simulink library "Lib_Piccolo"  (R2018b)
settings: Solver=VariableStepAuto  StartTime=0.0  StopTime=10.0  RelTol=1e-3
values from neighbouring files (symbols this model uses):
  AccelErrInt2Brakes = 0.15    [SimulationControlConfig16P.m]    (also in SimulationControlConfig16P_LEGACY.m; SimulationControlConfigTAILLESS.m = 0.2; SimulationControlConfigUTAIL.m = 0.2)
  AileronMax = 25    [SimulationControlConfig16P.m]    (also in SimulationControlConfig16P_LEGACY.m; SimulationControlConfigTAILLESS.m; SimulationControlConfigUTAIL.m)
  AileronPower = 0.00268    [SimulationControlConfig16P.m]    (also in SimulationControlConfig16P_LEGACY.m; SimulationControlConfigTAILLESS.m; SimulationControlConfigUTAIL.m)
  AileronSurfaceMax = 45    [SimulationControlConfig16P.m]    (also in SimulationControlConfig16P_LEGACY.m)
  AileronTrim = 0    [SimulationControlConfig16P.m]    (also in SimulationControlConfig16P_LEGACY.m; SimulationControlConfigTAILLESS.m; SimulationControlConfigUTAIL.m)
  Alt = 1000 + TerrainHeight    [SimulationStateConfig.m]
  AltCruise_m = testPlans(testIndx).terrainElevation * 0.3048 + 200    [SimulationControlConfig16P.m]    (also in SimulationControlConfigTAILLESS.m = 1083; SimulationControlConfigUTAIL.m = testPlans(testIndx).terrainElevation * 0.3048 + 152)
  AltitudeRate2PitchCmdIntegratorInit = 0.1    [SimulationControlPre.m]
  AltMax = 10000    [SimulationControlConfig16P.m]    (also in SimulationControlConfig16P_LEGACY.m; SimulationControlConfigTAILLESS.m; SimulationControlConfigUTAIL.m)
  AltMaxAccel = 1.25    [SimulationControlConfig16P.m]    (also in SimulationControlConfig16P_LEGACY.m = 0.9; SimulationControlConfigTAILLESS.m = 1.7; SimulationControlConfigUTAIL.m = 2)
  AltMin = 0    [SimulationControlConfig16P.m]    (also in SimulationControlConfig16P_LEGACY.m; SimulationControlConfigTAILLESS.m; SimulationControlConfigUTAIL.m)
  AltRateCmd2Pitch = 0.50    (= 0.5)    [SimulationControlConfig16P.m]    (also in SimulationControlConfig16P_LEGACY.m = 0.6; SimulationControlConfigTAILLESS.m = 0.2; SimulationControlConfigUTAIL.m = 0.3)
  AltRateError2Pitch = 0.40    (= 0.4)    [SimulationControlConfig16P.m]    (also in SimulationControlConfig16P_LEGACY.m; SimulationControlConfigTAILLESS.m = 0.55; SimulationControlConfigUTAIL.m = 0.55)
  AltRateErrorInt2Pitch = 0.50    (= 0.5)    [SimulationControlConfig16P.m]    (also in SimulationControlConfig16P_LEGACY.m = 0.45; SimulationControlConfigTAILLESS.m; SimulationControlConfigUTAIL.m = 0.75)
  AltRateLpfCutOff = 3    [SimulationControlConfig16P.m]    (also in SimulationControlConfig16P_LEGACY.m; SimulationControlConfigTAILLESS.m = 2; SimulationControlConfigUTAIL.m = 2)
  AutoNosegear2Rudder = 26    [SimulationControlConfig16P.m]    (also in SimulationControlConfig16P_LEGACY.m; SimulationControlConfigTAILLESS.m = 25.2; SimulationControlConfigUTAIL.m = 14)
  b = 5.54    [SimulationControlConfig16P.m]    (also in SimulationControlConfig16P_LEGACY.m; SimulationControlConfigTAILLESS.m = 2.37; SimulationControlConfigUTAIL.m = 2.37)
  Bank2AileronIntegratorInit = 0    [SimulationControlPre.m]
  BankMax_User = BankMax_User/180*pi    (= 0.523598775598)    [SimulationControlConfig16P.m]    (also in SimulationControlConfig16P_LEGACY.m; SimulationControlConfigTAILLESS.m = 0.610865238198; SimulationControlConfigUTAIL.m = 0.628318530718)
  baseLegFlaps = 20    [SimulationControlConfig16P.m]    (also in SimulationControlConfig16P_LEGACY.m = 0; SimulationControlConfigTAILLESS.m = 15; SimulationControlConfigUTAIL.m = 10)
  C = GeneticOpt.C    [SimulationCostFunction.m]
  c = Sw/b    (= 0.841696750903)    [SimulationControlConfig16P.m]    (also in SimulationControlConfig16P_LEGACY.m; SimulationControlConfigTAILLESS.m = 0.354008438819; SimulationControlConfigUTAIL.m = 0.354008438819)
  cell2WheelFactorMG = 5.98    [SimulationSensorConfig16P_LEGACY.m]
  cell2WheelFactorNG = 1    [SimulationSensorConfig16P_LEGACY.m]
  cellSatMaxMG = 15000    [SimulationSensorConfig16P.m]    (also in SimulationSensorConfig16P_LEGACY.m; SimulationSensorConfigTAILLESS7P.m; SimulationSensorConfigUTAIL7P.m)
  cellSatMaxNG = 1000    [SimulationSensorConfig16P.m]    (also in SimulationSensorConfig16P_LEGACY.m; SimulationSensorConfigTAILLESS7P.m; SimulationSensorConfigUTAIL7P.m)
  cellSatMinMG = -15000    [SimulationSensorConfig16P.m]    (also in SimulationSensorConfig16P_LEGACY.m; SimulationSensorConfigTAILLESS7P.m; SimulationSensorConfigUTAIL7P.m)
  cellSatMinNG = -1000    [SimulationSensorConfig16P.m]    (also in SimulationSensorConfig16P_LEGACY.m; SimulationSensorConfigTAILLESS7P.m; SimulationSensorConfigUTAIL7P.m)
  CL_Limit = CL_Max    (= 0.54)    [SimulationControlConfig16P.m]    (also in SimulationControlConfig16P_LEGACY.m; SimulationControlConfigTAILLESS.m; SimulationControlConfigUTAIL.m = 0.53)
  CL_Max = 0.54    [SimulationControlConfig16P.m]    (also in SimulationControlConfig16P_LEGACY.m; SimulationControlConfigTAILLESS.m; SimulationControlConfigUTAIL.m = 0.53)
  CL_Max_Nom = 0.465    [SimulationControlConfig16P.m]    (also in SimulationControlConfig16P_LEGACY.m; SimulationControlConfigTAILLESS.m = 0.39; SimulationControlConfigUTAIL.m)
  CL_Min = 0    [SimulationControlConfig16P.m]    (also in SimulationControlConfig16P_LEGACY.m; SimulationControlConfigTAILLESS.m; SimulationControlConfigUTAIL.m)
  ClimbMaxFraction = 0.35    [SimulationControlConfig16P.m]    (also in SimulationControlConfig16P_LEGACY.m = 0.24; SimulationControlConfigTAILLESS.m = 0.19; SimulationControlConfigUTAIL.m = 0.21)
  ClimboutMaxBank = 7.0    (= 7)    [SimulationControlConfig16P.m]    (also in SimulationControlConfig16P_LEGACY.m; SimulationControlConfigTAILLESS.m = 5; SimulationControlConfigUTAIL.m)
  ClimboutTimer = 7.0    (= 7)    [SimulationControlConfig16P.m]    (also in SimulationControlConfig16P_LEGACY.m; SimulationControlConfigTAILLESS.m; SimulationControlConfigUTAIL.m)
  dCl_per_dFlap = 0.005581818    [SimulationControlConfig16P.m]    (also in SimulationControlConfig16P_LEGACY.m = 0; SimulationControlConfigTAILLESS.m = 0; SimulationControlConfigUTAIL.m = 0)
  DecelerationCmd = 3.1    [SimulationControlConfig16P.m]    (also in SimulationControlConfig16P_LEGACY.m; SimulationControlConfigTAILLESS.m = 0.1; SimulationControlConfigUTAIL.m = 0.1)
  DeRotateLogicEndTimer = abs((NoseDownLimit_Deg-1)/DeRotateRamp_Dps)    [SimulationControlConfig16P.m]    (also in SimulationControlConfig16P_LEGACY.m; SimulationControlConfigTAILLESS.m; SimulationControlConfigUTAIL.m)
  DeRotateLogicHoldNoseUpTimer = 0.1    [SimulationControlConfig16P.m]    (also in SimulationControlConfig16P_LEGACY.m; SimulationControlConfigTAILLESS.m; SimulationControlConfigUTAIL.m)
  DeRotateLogicTimerTimeout = 2    [SimulationControlConfig16P.m]    (also in SimulationControlConfig16P_LEGACY.m; SimulationControlConfigTAILLESS.m; SimulationControlConfigUTAIL.m)
  DeRotateLowerCmdSaturation = 0    [SimulationControlConfig16P.m]    (also in SimulationControlConfig16P_LEGACY.m; SimulationControlConfigTAILLESS.m; SimulationControlConfigUTAIL.m)
  DeRotateRamp_Dps = 3    [SimulationControlConfig16P.m]    (also in SimulationControlConfig16P_LEGACY.m; SimulationControlConfigTAILLESS.m = 8; SimulationControlConfigUTAIL.m = 8)
  DeRotateUpperCmdSaturation = 7    [SimulationControlConfig16P.m]    (also in SimulationControlConfig16P_LEGACY.m; SimulationControlConfigTAILLESS.m; SimulationControlConfigUTAIL.m)
  DescentMaxFraction = 0.22    [SimulationControlConfig16P.m]    (also in SimulationControlConfig16P_LEGACY.m = 0.2; SimulationControlConfigTAILLESS.m = 0.17; SimulationControlConfigUTAIL.m = 0.17)
  DesktopSimTerrainOffset_m = 0.406    [SimulationAircraftConfig.m]
  downwindFlaps = 0    [SimulationControlConfig16P.m]    (also in SimulationControlConfig16P_LEGACY.m; SimulationControlConfigTAILLESS.m; SimulationControlConfigUTAIL.m)
  DP_init = 0.5*1.225*V_init^2    [SimulationControlConfig16P.m]    (also in SimulationControlConfig16P_LEGACY.m; SimulationControlConfigTAILLESS.m; SimulationControlConfigUTAIL.m)
  dscNoiseMG = 1    [SimulationSensorConfig16P_LEGACY.m]
  dscNoiseNG = 0.25    [SimulationSensorConfig16P_LEGACY.m]
  DSCnumBits = 24    [SimulationSensorConfig16P.m]    (also in SimulationSensorConfig16P_LEGACY.m; SimulationSensorConfigTAILLESS7P.m; SimulationSensorConfigUTAIL7P.m)
  DSCRangeMaxMG = 15000    [SimulationSensorConfig16P.m]    (also in SimulationSensorConfig16P_LEGACY.m; SimulationSensorConfigTAILLESS7P.m; SimulationSensorConfigUTAIL7P.m)
  DSCRangeMaxNG = 1000    [SimulationSensorConfig16P.m]    (also in SimulationSensorConfig16P_LEGACY.m; SimulationSensorConfigTAILLESS7P.m; SimulationSensorConfigUTAIL7P.m)
  DSCRangeMinMG = -15000    [SimulationSensorConfig16P.m]    (also in SimulationSensorConfig16P_LEGACY.m; SimulationSensorConfigTAILLESS7P.m; SimulationSensorConfigUTAIL7P.m)
  DSCRangeMinNG = -1000    [SimulationSensorConfig16P.m]    (also in SimulationSensorConfig16P_LEGACY.m; SimulationSensorConfigTAILLESS7P.m; SimulationSensorConfigUTAIL7P.m)
  dt = DLLSim.dt    [SimulationTimeStep.m]    (also in SimulationTrim.m = 0.02)
  EarlyTouchdownThreshold = 3.0    (= 3)    [SimulationControlConfig16P.m]    (also in SimulationControlConfig16P_LEGACY.m; SimulationControlConfigTAILLESS.m = 2.2; SimulationControlConfigUTAIL.m = 2.5)
  ElevatorDeflectionRate = 15    [SimulationControlConfig16P.m]    (also in SimulationControlConfig16P_LEGACY.m = 12; SimulationControlConfigTAILLESS.m = 10; SimulationControlConfigUTAIL.m = 12)
  ElevatorMax = 25    [SimulationControlConfig16P.m]    (also in SimulationControlConfig16P_LEGACY.m; SimulationControlConfigTAILLESS.m; SimulationControlConfigUTAIL.m)
  ElevatorPower = -0.002209    [SimulationControlConfig16P.m]    (also in SimulationControlConfig16P_LEGACY.m; SimulationControlConfigTAILLESS.m = -0.002956; SimulationControlConfigUTAIL.m = -0.00205983)
  ElevatorTrim = -3.5    [SimulationControlConfig16P.m]    (also in SimulationControlConfig16P_LEGACY.m; SimulationControlConfigTAILLESS.m = -6; SimulationControlConfigUTAIL.m = -8)
  elevonBias = 0    [SimulationControlConfig16P.m]    (also in SimulationControlConfig16P_LEGACY.m; SimulationControlConfigTAILLESS.m; SimulationControlConfigUTAIL.m)
  Enable_TAS_Protection = 0    [SimulationControlConfig16P.m]    (also in SimulationControlConfig16P_LEGACY.m; SimulationControlConfigTAILLESS.m; SimulationControlConfigUTAIL.m)
  EnableCrossTrackAbort = 1    [SimulationControlConfig16P.m]    (also in SimulationControlConfigTAILLESS.m; SimulationControlConfigUTAIL.m)
  EnergyBandwidth = 0.02    [SimulationControlConfig16P.m]    (also in SimulationControlConfig16P_LEGACY.m; SimulationControlConfigTAILLESS.m = 0.06; SimulationControlConfigUTAIL.m = 0.06)
  EngineLhFuelCut = 0    [SimulationAircraftConfig.m]
  EngineRhFuelCut = 0    [SimulationAircraftConfig.m]
  FastThrottleRate = 0.075    [SimulationControlConfig16P.m]    (also in SimulationControlConfig16P_LEGACY.m = 0.05; SimulationControlConfigTAILLESS.m = 0.1; SimulationControlConfigUTAIL.m = 0.1)
  FilterWarmUpTime = 2    [SimulationSensorConfig16P.m]    (also in SimulationSensorConfig16P_LEGACY.m; SimulationSensorConfigTAILLESS7P.m; SimulationSensorConfigUTAIL7P.m)
  finalApproachFlaps = 20    [SimulationControlConfig16P.m]    (also in SimulationControlConfig16P_LEGACY.m = 0; SimulationControlConfigTAILLESS.m = 22; SimulationControlConfigUTAIL.m = 10)
  FinalDescentSlope_Deg = testPlans(testIndx).descentSlope    [SimulationControlConfig16P.m]    (also in SimulationControlConfig16P_LEGACY.m; SimulationControlConfigTAILLESS.m; SimulationControlConfigUTAIL.m)
  flapMax = 0    [SimulationControlConfig16P.m]    (also in SimulationControlConfig16P_LEGACY.m; SimulationControlConfigTAILLESS.m; SimulationControlConfigUTAIL.m)
  flapRate = 7.5    [SimulationControlConfig16P.m]    (also in SimulationControlConfig16P_LEGACY.m; SimulationControlConfigTAILLESS.m = 6.6; SimulationControlConfigUTAIL.m)
  FlareHeight = 5    [SimulationControlConfig16P.m]    (also in SimulationControlConfig16P_LEGACY.m = 4.8; SimulationControlConfigTAILLESS.m = 2.5; SimulationControlConfigUTAIL.m = 2)
  FlareVerticalRate_mps = -0.4    [SimulationControlConfig16P.m]    (also in SimulationControlConfig16P_LEGACY.m = -0.5; SimulationControlConfigTAILLESS.m = -0.15; SimulationControlConfigUTAIL.m = -0.15)
  Fp_Aileron = 0.55*2*pi*RollRateLpfCutoff*dt    [SimulationControlConfig16P.m]    (also in SimulationControlConfig16P_LEGACY.m; SimulationControlConfigTAILLESS.m; SimulationControlConfigUTAIL.m)
  Fp_Alt = 0.55*AltBandwidth    (= 0.099)    [SimulationControlConfig16P.m]    (also in SimulationControlConfig16P_LEGACY.m; SimulationControlConfigTAILLESS.m = 0.587477826221; SimulationControlConfigUTAIL.m = 0.69115038379)
  Fp_AltRate = 0.55*2*pi*AltRateLpfCutOff*dt    [SimulationControlConfig16P.m]    (also in SimulationControlConfig16P_LEGACY.m; SimulationControlConfigTAILLESS.m; SimulationControlConfigUTAIL.m)
  Fp_Elevator = 0.55*2*pi*PitchRateLpfCutoff*dt    [SimulationControlConfig16P.m]    (also in SimulationControlConfig16P_LEGACY.m; SimulationControlConfigTAILLESS.m; SimulationControlConfigUTAIL.m)
  Fp_Energy = 0.55*2*pi*EnergyBandwidth    (= 0.069115038379)    [SimulationControlConfig16P.m]    (also in SimulationControlConfig16P_LEGACY.m; SimulationControlConfigTAILLESS.m = 0.207345115137; SimulationControlConfigUTAIL.m = 0.207345115137)
  Fp_Energy2 = 0.55*2*pi*EnergyBandwidth*dt    [SimulationControlConfig16P.m]    (also in SimulationControlConfig16P_LEGACY.m; SimulationControlConfigTAILLESS.m; SimulationControlConfigUTAIL.m)
  Fp_Pitch = 0.55*2*pi*PitchBandwidth    (= 2.76460153516)    [SimulationControlConfig16P.m]    (also in SimulationControlConfig16P_LEGACY.m = 3.11017672705; SimulationControlConfigTAILLESS.m = 3.80132711084; SimulationControlConfigUTAIL.m = 2.41902634326)
  Fp_Pitch_2 = 0.55*2*pi*PitchBandwidth*dt    [SimulationControlConfig16P.m]    (also in SimulationControlConfig16P_LEGACY.m; SimulationControlConfigTAILLESS.m; SimulationControlConfigUTAIL.m)
  Fp_Roll = RollBandwidth^2    (= 1)    [SimulationControlConfig16P.m]    (also in SimulationControlConfig16P_LEGACY.m = 1.44; SimulationControlConfigTAILLESS.m; SimulationControlConfigUTAIL.m)
  Fp_Rudder = 0.55*2*pi*YawRateLpfCutoff*dt    [SimulationControlConfig16P.m]    (also in SimulationControlConfig16P_LEGACY.m; SimulationControlConfigTAILLESS.m; SimulationControlConfigUTAIL.m)
  Fp_TAS = 0.55*2*pi*TASBandwidth    (= 0.103672557568)    [SimulationControlConfig16P.m]    (also in SimulationControlConfig16P_LEGACY.m; SimulationControlConfigTAILLESS.m = 0.172787595947; SimulationControlConfigUTAIL.m = 0.172787595947)
  Fp_TAS_Filter = 2*pi*TasLpfCutoff*dt    [SimulationControlConfig16P.m]    (also in SimulationControlConfig16P_LEGACY.m; SimulationControlConfigTAILLESS.m; SimulationControlConfigUTAIL.m)
  Fp_Turn = 0.55*2*pi*TurnErrLPFcutoff    (= 0.0345575191895)    [SimulationControlConfig16P.m]    (also in SimulationControlConfig16P_LEGACY.m; SimulationControlConfigTAILLESS.m = 0.172787595947; SimulationControlConfigUTAIL.m = 0.172787595947)
  Fp_TurnDerr = 0.55*2*pi*TurnDerivativeLPFcutoff    (= 0.0345575191895)    [SimulationControlConfig16P.m]    (also in SimulationControlConfig16P_LEGACY.m; SimulationControlConfigTAILLESS.m = 0.172787595947; SimulationControlConfigUTAIL.m = 0.172787595947)
  FTV = 3    [SimulationAircraftConfig.m]
  ftvStaticPositionError = 1/1.18    (= 0.847457627119)    [SimulationSensorConfig16P.m]    (also in SimulationSensorConfig16P_LEGACY.m; SimulationSensorConfigTAILLESS7P.m = 1; SimulationSensorConfigUTAIL7P.m = 1)
  g = 9.81    [SimulationStateConfig.m]
  GustSpd_Kts = testPlans(testIndx).gustSpd    [SimulationStateConfig.m]
  GustTriggerVal = testPlans(testIndx).gustTriggerVal    [SimulationStateConfig.m]
  HeadingErr2TurnRate = 0.5    [SimulationControlConfig16P.m]    (also in SimulationControlConfig16P_LEGACY.m; SimulationControlConfigTAILLESS.m; SimulationControlConfigUTAIL.m)
  HeadingErrDer2TurnRate = 0.3    [SimulationControlConfig16P.m]    (also in SimulationControlConfig16P_LEGACY.m; SimulationControlConfigTAILLESS.m; SimulationControlConfigUTAIL.m)
  IASbounce = IASstall*0.8    [SimulationControlPre.m]
  IAScruiseCMD = sqrt(2*m*9.81/(1.225*Sw*CL_cruise))    [SimulationControlConfig16P.m]    (also in SimulationControlConfig16P_LEGACY.m; SimulationControlConfigTAILLESS.m; SimulationControlConfigUTAIL.m)
  IASfinalCMD = 1.12 * IASmin    [SimulationControlConfig16P.m]    (also in SimulationControlConfig16P_LEGACY.m = 1.10 * IASmin; SimulationControlConfigTAILLESS.m = 1.10 * IASmin; SimulationControlConfigUTAIL.m = 1.15 * IASmin)
  IASflareCMD = IASstall    [SimulationControlConfig16P.m]    (also in SimulationControlConfig16P_LEGACY.m; SimulationControlConfigTAILLESS.m; SimulationControlConfigUTAIL.m)
  IASmax = 64    [SimulationControlConfig16P.m]    (also in SimulationControlConfig16P_LEGACY.m = 46; SimulationControlConfigTAILLESS.m = 38.58; SimulationControlConfigUTAIL.m = 35)
  IASmin = sqrt(2*m*9.81/(1.225*Sw*0.9*CL_Max_Nom))    [SimulationControlConfig16P.m]    (also in SimulationControlConfig16P_LEGACY.m; SimulationControlConfigTAILLESS.m; SimulationControlConfigUTAIL.m)
  IASshortCMD = IASstall    [SimulationControlConfig16P.m]    (also in SimulationControlConfig16P_LEGACY.m; SimulationControlConfigTAILLESS.m; SimulationControlConfigUTAIL.m)
  IASstall = sqrt(2*m*9.81/(1.225*Sw*CL_Max))    [SimulationControlConfig16P.m]    (also in SimulationControlConfig16P_LEGACY.m; SimulationControlConfigTAILLESS.m; SimulationControlConfigUTAIL.m)
  inFlight = 1    [SimulationControlConfig16P.m]    (also in SimulationControlConfigTAILLESS.m; SimulationControlConfigUTAIL.m)
  JetCatOffset = 5    [SimulationControlConfig16P.m]    (also in SimulationControlConfig16P_LEGACY.m)
  LaunchRollingElevator = -1.5    [SimulationControlConfig16P.m]    (also in SimulationControlConfig16P_LEGACY.m; SimulationControlConfigTAILLESS.m = 1; SimulationControlConfigUTAIL.m = 1)
  ldg_NosegearMax = 10    [SimulationControlConfig16P.m]    (also in SimulationControlConfig16P_LEGACY.m; SimulationControlConfigTAILLESS.m; SimulationControlConfigUTAIL.m)
  ldg_TrackVyErrInt2Nosegear = 0.1250    (= 0.125)    [SimulationControlConfig16P.m]    (also in SimulationControlConfig16P_LEGACY.m; SimulationControlConfigTAILLESS.m = 0.00714285714286; SimulationControlConfigUTAIL.m = 0.00714285714286)
  ldg_TrackVyErrPro2Nosegear = 0.35    [SimulationControlConfig16P.m]    (also in SimulationControlConfig16P_LEGACY.m; SimulationControlConfigTAILLESS.m = 0.0546666666667; SimulationControlConfigUTAIL.m = 0.0546666666667)
  ldg_TrackY2Vy = 0.07    [SimulationControlConfig16P.m]    (also in SimulationControlConfig16P_LEGACY.m; SimulationControlConfigTAILLESS.m = 0.17; SimulationControlConfigUTAIL.m = 0.17)
  ldg_Vy2NosegearScalingPower = 1.075    [SimulationControlConfig16P.m]    (also in SimulationControlConfig16P_LEGACY.m; SimulationControlConfigTAILLESS.m = 0.6; SimulationControlConfigUTAIL.m = 0.5)
  ldg_Y2VyScalingPower = 0.175    [SimulationControlConfig16P.m]    (also in SimulationControlConfig16P_LEGACY.m; SimulationControlConfigTAILLESS.m = 0; SimulationControlConfigUTAIL.m = 0)
  ldg_YawRate2Nosegear = 0.175    [SimulationControlConfig16P.m]    (also in SimulationControlConfig16P_LEGACY.m; SimulationControlConfigTAILLESS.m = 0.065; SimulationControlConfigUTAIL.m = 0.065)
  LiftSlope = 0.064285    [SimulationControlConfig16P.m]    (also in SimulationControlConfig16P_LEGACY.m; SimulationControlConfigTAILLESS.m = 0.058631; SimulationControlConfigUTAIL.m)
  LPFaileronInit = 0    [SimulationControlPre.m]
  LPFclestInit = 0    [SimulationControlPre.m]
  LPFenergyFFInit = 0    [SimulationControlPre.m]
  LPFtasInit = V_init + 2    [SimulationControlPre.m]
  LPFthrottleInit = ThrottleTrim    [SimulationControlPre.m]
  LPFturnErrInit = 0    [SimulationControlPre.m]
  ... (+115 more)
undefined symbols (not defined in the file or in its folder): abortFlag, alphaHPF, apmDelay, BRWNOUT, CRAWOR, CRAWUR, DiscIntNeverNeededParam, DLLSim, DLLSimStep, ECOMOR, ECOMUR, Fp_Tas, GustTrigger_HeightAgl_m, IPSTAT, LCINTEG, Ldg_Persist_Time, LOWER_FLAGS, MSG_ENABLE, NoiseStd, OLDVAL, OVERRIDE_ENABLE, OVERRIDE_VALUE, REBOOT, reversionEnable, revIASMax, revIASMin, revPitchMax, revPitchMin, revPitchRateMax, revRollMax, revRollRateMax, SAMPLE, SCALON, SensorModel, sigbuilder_block, Sim_Vx, Sim_Vy, Sim_Vz, Sim_Xpos, Sim_Ypos, Sim_Zpos, SYSOR, SYSUR, TARE, TEMPOR, TEMPUR, testIndx, testPlan, testPlans, Trim_piccoloInCmd, Trim_REFSI_FD_IN_nmodeCgShifterCmd_Ft, Trim_REFSI_FD_IN_nmodeFlapLhIBCmd_Deg, Trim_REFSI_FD_IN_nmodeFlapLhOBCmd_Deg, Trim_REFSI_FD_IN_nmodeFlapRhIBCmd_Deg, Trim_REFSI_FD_IN_nmodeFlapRhOBCmd_Deg, Trim_REFSI_FD_IN_nmodeSlatLhCmd_Deg, Trim_REFSI_FD_IN_nmodeSlatRhCmd_Deg, Trim_REFSI_FD_IN_nmodeSplrLhInbdCmd_Deg, Trim_REFSI_FD_IN_nmodeSplrLhOutbdCmd_Deg ... (+5)
libraries: simulink x866, aerolibconvert2 x60, $bdroot x52, aerolibatmos2 x5, dspswit3 x5, simulink_extras x4, dsparch4 x2, Lib_Piccolo_Alt x2, eeGeneralControl x1, dspindex x1
(part 13 of 44)

== system Lib_Piccolo/Pitch to Elevator/LPF Elevator ==
  Input : Inport
  Reset : Inport  Port=2
  ResetValue : Inport  Port=3
  Add1 : Sum  Inputs=++|
  Compare To Constant2 : simulink/Logic and Bit Operations/Compare To Constant  relop=>  const=0  OutDataTypeStr=uint8
  Constant11 : Constant  Value=PitchRateLpfCutoff
  Switch : Switch  Criteria=u2 > Threshold
  Switch1 : Switch  Criteria=u2 > Threshold
  Unit Delay1 : UnitDelay  InitialCondition=LPFvRate2PitchInit*pi/180  SampleTime=-1
  a1 : Gain  Gain=1-Fp_Elevator
  b0 : Gain  Gain=Fp_Elevator
  Output : Outport
  wires:
  ResetValue/1 -> Switch/1
  Reset/1 -> Switch/2
  Switch/1 -> Unit Delay1/1
  Input/1 -> b0/1, Switch1/3
  Add1/1 -> Switch1/1, Switch/3
  b0/1 -> Add1/2
  Unit Delay1/1 -> a1/1
  a1/1 -> Add1/1
  Switch1/1 -> Output/1
  Compare To Constant2/1 -> Switch1/2
  Constant11/1 -> Compare To Constant2/1

== system Lib_Piccolo/Pitch to Elevator/Pitch Moment Caused By Damping ==
  note: An estimation of damping moment produced proportionally to body pitch rate.
  PitchRate_Body : Inport
  TAS : Inport  Port=2
  AverageWingChord : Constant  Value=c
  Constant : Constant  Value=PitchDamping
  Gain : Gain  Gain=2
  Multiply : Product  Inputs=***/
  DAMP : Outport
  wires:
  PitchRate_Body/1 -> Multiply/2
  TAS/1 -> Gain/1
  Constant/1 -> Multiply/1
  Multiply/1 -> DAMP/1
  Gain/1 -> Multiply/4
  AverageWingChord/1 -> Multiply/3

== system Lib_Piccolo/Pitch to Elevator/Reference Frame Conversion and Pitch Rate Limit Determination ==
  PitchCmd_Euler : Inport
  Pitch_Euler : Inport  Port=2
  Roll_Euler : Inport  Port=3
  V : Inport  Port=4
  Q : Inport  Port=5
  AeroVsStruct_Limit : Subsystem
  Constant : Constant  Value=PitchRateMax_User
  MATLAB Function : MATLAB Function  TreatAsAtomicUnit=on
  Saturation : Saturate  UpperLimit=100  LowerLimit=5
  Terminator : Terminator
  Terminator1 : Terminator
  PitchCmd_Body : Outport
  "Pitch_Body " : Outport  Port=2
  "Scalar " : Outport  Port=3
  PitchRateCmd_Body : Outport  Port=4
  "PitchRateLimit_Max " : Outport  Port=5
  "PitchRateLimit_Min " : Outport  Port=6
  wires:
  MATLAB Function/8(nPrime_Min) -> Terminator1/1
  MATLAB Function/7(nPrime_Max) -> Terminator/1
  Q/1 -> AeroVsStruct_Limit/1(Q)
  AeroVsStruct_Limit/2("nMin ") -> MATLAB Function/6(nMin)
  AeroVsStruct_Limit/1(nMax) -> MATLAB Function/5(nMax)
  MATLAB Function/4(PitchRateCmd_Body) -> PitchRateCmd_Body/1
  Constant/1 -> MATLAB Function/7(PitchRateMax_User)
  MATLAB Function/6(PitchRateLimit_Min) -> "PitchRateLimit_Min "/1
  MATLAB Function/5(PitchRateLimit_Max) -> "PitchRateLimit_Max "/1
  MATLAB Function/3(Scalar) -> "Scalar "/1
  MATLAB Function/2(Pitch_Body) -> "Pitch_Body "/1
  MATLAB Function/1(PitchCmd_Body) -> PitchCmd_Body/1
  Roll_Euler/1 -> MATLAB Function/3(Roll_Euler)
  Pitch_Euler/1 -> MATLAB Function/2(Pitch_Euler)
  PitchCmd_Euler/1 -> MATLAB Function/1(PitchCmd_Euler)
  V/1 -> Saturation/1
  Saturation/1 -> MATLAB Function/4(V)

== system Lib_Piccolo/Pitch to Elevator/TASLimit ==
  note: TAS saturates at ~ 100mps which in IAS is 6125Pa
  apMode : Inport
  <V_mps> : Inport  Port=2
  Compare To Constant1 : simulink/Logic and Bit Operations/Compare To Constant  relop=>=  const=5  OutDataTypeStr=uint8
  Compare To Constant2 : simulink/Logic and Bit Operations/Compare To Constant  relop=>=  const=11  OutDataTypeStr=uint8
  Compare To Constant4 : simulink/Logic and Bit Operations/Compare To Constant  relop=>=  const=10  OutDataTypeStr=uint8
  Gain : Gain  Gain=0.8
  Latch : Subsystem
  Saturation Dynamic1 : simulink/Discontinuities/Saturation Dynamic  OutMin=[]  OutMax=[]  OutDataTypeStr=Inherit: Same as second input  OutDataType=fixdt(1, 16)  OutScaling=2^-10  DoSatur=off
  Switch1 : Switch  Criteria=u2 > Threshold
  Switch2 : Switch  Criteria=u2 > Threshold
  TASmax : Constant  Value=100
  Out1 : Outport
  wires:
  TASmax/1 -> Saturation Dynamic1/1
  Gain/1 -> Switch2/1  "IASbounce"
  Compare To Constant1/1 -> Latch/2(Enable/!Rst)
  Switch1/1 -> Switch2/3
  apMode/1 -> Compare To Constant4/1, Compare To Constant2/1, Compare To Constant1/1
  Compare To Constant2/1 -> Latch/1(D)
  Latch/1(Q_Latched) -> Switch2/2
  <V_mps>/1 -> Saturation Dynamic1/2
  [IASmin] -> Switch1/3
  Saturation Dynamic1/1 -> Out1/1
  [IASstall] -> Switch1/1, Gain/1
  Compare To Constant4/1 -> Switch1/2
  Switch2/1 -> Saturation Dynamic1/3

== system Lib_Piccolo/Pitch to Elevator/Triggered Subsystem ==
  In1 : Inport
  Trigger : TriggerPort  TriggerType=falling  VariantControl=Variant
  Out1 : Outport
  wires:
  In1/1 -> Out1/1

== system Lib_Piccolo/Pitch to Elevator/resetCondition ==
  Compare To Constant1 : simulink/Logic and Bit Operations/Compare To Constant  relop=<=  const=2  OutDataTypeStr=uint8
  Compare To Constant3 : simulink/Logic and Bit Operations/Compare To Constant  relop===  const=11  OutDataTypeStr=uint8
  NOT : Logic  Operator=NOT  IconShape=distinctive  AllPortsSameDT=off  OutDataTypeStr=boolean
  OR : Logic  Operator=OR  Inputs=3  IconShape=distinctive  AllPortsSameDT=off  OutDataTypeStr=boolean
  reset : Outport
  wires:
  NOT/1 -> OR/3
  [ApGlobal] -> NOT/1
  Compare To Constant1/1 -> OR/2
  OR/1 -> reset/1  "Sim.KI_Pitch_Reset"
  Compare To Constant3/1 -> OR/1
  [Pic_AP_Mode] -> Compare To Constant3/1, Compare To Constant1/1

== system Lib_Piccolo/Pitch to Elevator/resetVal ==
  note: This init value is intended to aid trimming at start of in-flight simulation and should not be used for reset during liftoffs/bouncing. Will use 0 as alternative reset value as was done previously
  Constant1 : Constant  Value=Pitch2ElevatorIntegratorInit
  Constant2 : Constant  Value=0
  Constant3 : Constant  Value=0
  Switch : Switch  Threshold=9
  Switch1 : Switch  Threshold=3
  resetVal : Outport
  wires:
  Constant3/1 -> Switch1/3
  Switch1/1 -> Switch/3
  Constant1/1 -> Switch1/1
  Switch/1 -> resetVal/1
  [Pic_AP_Mode] -> Switch/2, Switch1/2
  Constant2/1 -> Switch/1

== system Lib_Piccolo/REF INS Replay/Slope Vz Calculation ==
  VGround : Inport
  apMode : Inport  Port=2
  Compare To Constant : simulink/Logic and Bit Operations/Compare To Constant  relop=>=  const=5  OutDataTypeStr=boolean
  Compare To Constant1 : simulink/Logic and Bit Operations/Compare To Constant  relop=>=  const=9  OutDataTypeStr=boolean
  Constant13 : Constant  Value=FinalDescentSlope_Deg*pi/180
  Constant14 : Constant  Value=ShortDescentSlope_Deg*pi/180
  CruiseSlope_Deg : Constant  Value=0
  Gain : Gain  Gain=-1
  Multiply10 : Product
  Sin3 : Trigonometry
  Switch3 : Switch  Criteria=u2 > Threshold
  Switch4 : Switch  Criteria=u2 > Threshold
  Vz_Cmd : Outport
  wires:
  Compare To Constant/1 -> Switch4/2
  Compare To Constant1/1 -> Switch3/2
  Switch4/1 -> Sin3/1
  Gain/1 -> Multiply10/1
  Constant13/1 -> Switch3/3
  VGround/1 -> Gain/1
  CruiseSlope_Deg/1 -> Switch4/3
  Multiply10/1 -> Vz_Cmd/1
  Constant14/1 -> Switch3/1
  Sin3/1 -> Multiply10/2
  Switch3/1 -> Switch4/1
  apMode/1 -> Compare To Constant1/1, Compare To Constant/1

== system Lib_Piccolo/Steering Controller Landing/Nosegear rudder mixer  ==
  "Desired nosegear " : Inport
  NoseGear2Rudder : Gain  Gain=AutoNosegear2Rudder
  Saturation : Saturate  UpperLimit=ldg_NosegearMax  LowerLimit=-ldg_NosegearMax
  Saturation1 : Saturate  UpperLimit=RudderMax  LowerLimit=-RudderMax
  rad2deg : Gain  Gain=180/pi
  Nosegear command : Outport
  Rudder command : Outport  Port=2
  wires:
  rad2deg/1 -> Saturation/1, NoseGear2Rudder/1
  "Desired nosegear "/1 -> rad2deg/1
  NoseGear2Rudder/1 -> Saturation1/1
  Saturation/1 -> Nosegear command/1
  Saturation1/1 -> Rudder command/1

== system Lib_Piccolo/Steering Controller Landing/Nosegear scaling based on ground speed ==
  Ground Speed : Inport
  "Vy to nosegear scaling " : Inport  Port=2
  Divide : Product  Inputs=*/
  SteeringArm : Constant  Value=SteeringArm
  Vy Scalar1 : Math  Operator=pow  SaturateOnIntegerOverflow=on
  nosegear scalar : Outport
  wires:
  "Vy to nosegear scaling "/1 -> Vy Scalar1/2
  Divide/1 -> nosegear scalar/1
  SteeringArm/1 -> Divide/1
  Vy Scalar1/1 -> Divide/2
  Ground Speed/1 -> Vy Scalar1/1

== system Lib_Piccolo/Steering Controller Landing/Vy scaling based on ground speed ==
  Ground Speed : Inport
  Y to Vy scaling power : Inport  Port=2
  Power Function : Math  Operator=pow  SaturateOnIntegerOverflow=on
  Vy Scalar : Outport
  wires:
  Y to Vy scaling power/1 -> Power Function/2
  Ground Speed/1 -> Power Function/1
  Power Function/1 -> Vy Scalar/1

== system Lib_Piccolo/Steering Controller Transition/Nosegear rudder mixer  ==
  "Desired nosegear " : Inport
  NoseGear2Rudder : Gain  Gain=AutoNosegear2Rudder
  Saturation : Saturate  UpperLimit=NosegearMax  LowerLimit=-NosegearMax
  Saturation1 : Saturate  UpperLimit=RudderMax  LowerLimit=-RudderMax
  rad2deg : Gain  Gain=180/pi
  Nosegear command : Outport
  Rudder command : Outport  Port=2
  wires:
  rad2deg/1 -> Saturation/1, NoseGear2Rudder/1
  "Desired nosegear "/1 -> rad2deg/1
  NoseGear2Rudder/1 -> Saturation1/1
  Saturation/1 -> Nosegear command/1
  Saturation1/1 -> Rudder command/1

== system Lib_Piccolo/Steering Controller Transition/Nosegear scaling based on ground speed ==
  Ground Speed : Inport
  "Vy to nosegear scaling " : Inport  Port=2
  Divide : Product  Inputs=*/
  SteeringArm : Constant  Value=SteeringArm
  Vy Scalar1 : Math  Operator=pow  SaturateOnIntegerOverflow=on
  nosegear scalar : Outport
  wires:
  "Vy to nosegear scaling "/1 -> Vy Scalar1/2
  Divide/1 -> nosegear scalar/1
  SteeringArm/1 -> Divide/1
  Vy Scalar1/1 -> Divide/2
  Ground Speed/1 -> Vy Scalar1/1

== system Lib_Piccolo/Steering Controller Transition/Vy scaling based on ground speed ==
  Ground Speed : Inport
  Y to Vy scaling power : Inport  Port=2
  Power Function : Math  Operator=pow  SaturateOnIntegerOverflow=on
  Vy Scalar : Outport
  wires:
  Y to Vy scaling power/1 -> Power Function/2
  Ground Speed/1 -> Power Function/1
  Power Function/1 -> Vy Scalar/1

== system Lib_Piccolo/Throttle Control (Airspeed Mode)/1st Order Reference Model ==
  Pcmd : Inport
  Vcmd : Inport  Port=2
  Pact : Inport  Port=3
  "V " : Inport  Port=4
  Constant : Constant  Value=0
  Gain : Gain  Gain=Fp_Energy
  Gain3 : Gain  Gain=m*g
  Gain4 : Gain  Gain=m*g
  Saturation Dynamic : simulink/Discontinuities/Saturation Dynamic  OutMin=[]  OutMax=[]  OutDataTypeStr=Inherit: Same as second input  OutDataType=fixdt(1, 16)  OutScaling=2^-10  DoSatur=off
  Scope : Scope
  Subsystem : Subsystem
  Sum : Sum  Inputs=|+-
  Sum1 : Sum  Inputs=|++
  Rf : Outport
  wires:
  Saturation Dynamic/1 -> Rf/1  "Rf"
  Pcmd/1 -> Sum/1
  Pact/1 -> Sum/2
  Sum/1 -> Scope/1, Gain/1
  Gain/1 -> Sum1/2
  Sum1/1 -> Saturation Dynamic/2
  Constant/1 -> Sum1/1
  Vcmd/1 -> Subsystem/2(Vcmd)
  Subsystem/2("hdotMin ") -> Gain4/1
  Subsystem/1(hdotMax) -> Gain3/1
  "V "/1 -> Subsystem/1(V)
  Gain3/1 -> Saturation Dynamic/1
  Gain4/1 -> Saturation Dynamic/3

== system Lib_Piccolo/Throttle Control (Airspeed Mode)/Subsystem ==
  Throttle In : Inport
  Reset LPF : Inport  Port=2
  LPF Throttle Alpha : Subsystem
  Throttle Out : Outport
  wires:
  LPF Throttle Alpha/1(Output) -> Throttle Out/1  "TLA"
  Reset LPF/1 -> LPF Throttle Alpha/2(Reset)
  Throttle In/1 -> LPF Throttle Alpha/1(Input)  "TLA_Prefilter"

== system Lib_Piccolo/Throttle Control (Alt Mode)/1st Order Reference Model ==
  Pcmd : Inport
  Pact : Inport  Port=2
  "V " : Inport  Port=3
  Constant : Constant  Value=0
  Gain : Gain  Gain=Fp_Energy
  Gain1 : Gain  Gain=m*TASRateMax
  Gain2 : Gain  Gain=-1
  Saturation Dynamic : simulink/Discontinuities/Saturation Dynamic  OutMin=[]  OutMax=[]  OutDataTypeStr=Inherit: Same as second input  OutDataType=fixdt(1, 16)  OutScaling=2^-10  DoSatur=off
  Sum : Sum  Inputs=|+-
  Sum1 : Sum  Inputs=|++
  TEC Ref Max Rate Limit : Subsystem  Commented=on
  Rf : Outport
  wires:
  Saturation Dynamic/1 -> Rf/1  "Rf"
  Pcmd/1 -> Sum/1
  Pact/1 -> Sum/2
  Sum/1 -> Gain/1
  Gain/1 -> Sum1/2
  Sum1/1 -> Saturation Dynamic/2
  Gain1/1 -> Saturation Dynamic/1, Gain2/1
  Gain2/1 -> Saturation Dynamic/3
  Constant/1 -> Sum1/1
  "V "/1 -> Gain1/1

== system Lib_Piccolo/Throttle Control (Alt Mode)/Filter and Throttle Cut ==
  note: If IASFlareCMD equal 0 and Piccolo in Flare State Set Engine to Idle
  note: Set Engine To Idle After Touchdown
  Throttle In : Inport
  Reset LPF : Inport  Port=2
  apMode : Inport  Port=3
  Throttle Ramp In : Inport  Port=4
  AND : Logic  IconShape=distinctive  AllPortsSameDT=off  OutDataTypeStr=boolean
  Compare To Constant1 : simulink/Logic and Bit Operations/Compare To Constant  relop=>=  const=10  OutDataTypeStr=boolean
  Compare To Constant2 : simulink/Logic and Bit Operations/Compare To Constant  relop=>=  const=11  OutDataTypeStr=boolean
  Compare To Constant3 : simulink/Logic and Bit Operations/Compare To Constant  relop=<=  const=3  OutDataTypeStr=boolean
  Compare To Constant4 : simulink/Logic and Bit Operations/Compare To Constant  relop===  const=0  OutDataTypeStr=boolean
  Constant8 : Constant  Value=-ThrottleRateMax
  Constant9 : Constant  Value=IASflareCMD
  Discrete-Time Integrator1 : DiscreteIntegrator  ExternalReset=rising  InitialConditionSource=external  SampleTime=-1  LimitOutput=on  UpperSaturationLimit=ThrottleMax  LowerSaturationLimit=ThrottleMin  ICPrevOutput=DiscIntNeverNeededParam  ICPrevScaledInput=DiscIntNeverNeededParam
  LPF Throttle Alpha : Subsystem
  OR : Logic  Operator=OR  IconShape=distinctive  AllPortsSameDT=off  OutDataTypeStr=boolean
  OR1 : Logic  Operator=OR  IconShape=distinctive  AllPortsSameDT=off  OutDataTypeStr=boolean
  Switch : Switch  Criteria=u2 > Threshold
  Switch1 : Switch  Criteria=u2 > Threshold
  Switch8 : Switch  Criteria=u2 > Threshold
  Unit Delay : UnitDelay  SampleTime=-1
  Throttle Out : Outport
  wires:
  Compare To Constant4/1 -> AND/2
  Compare To Constant1/1 -> AND/1
  OR/1 -> Discrete-Time Integrator1/2, Switch8/2, Switch1/2, OR1/2
  AND/1 -> OR/1
  Constant9/1 -> Compare To Constant4/1
  Switch8/1 -> Throttle Out/1  "TLA"
  Throttle In/1 -> Switch1/3  "TLA_PreFilter"
  Compare To Constant2/1 -> OR/2
  Reset LPF/1 -> OR1/1
  apMode/1 -> Compare To Constant2/1, Compare To Constant3/1, Compare To Constant1/1
  LPF Throttle Alpha/1(Output) -> Switch/3, Switch8/3  "TLA_Postfilter"
  Constant8/1 -> Discrete-Time Integrator1/1
  Discrete-Time Integrator1/1 -> Switch8/1, Switch1/1  "Sim.TLA_Ramp"
  OR1/1 -> LPF Throttle Alpha/2(Reset)
  Switch1/1 -> LPF Throttle Alpha/1(Input)  "TLA"
  Throttle Ramp In/1 -> Switch/1
  Unit Delay/1 -> Discrete-Time Integrator1/3
  Compare To Constant3/1 -> Switch/2
  Switch/1 -> Unit Delay/1

== system Lib_Piccolo/Throttle Control (Alt Mode)/Flare Throttle Modifications 2 ==
  Throttle In (0 - 100%) : Inport
  Piccolo Elevator In (deg.) : Inport  Port=2
  AP Mode (0 - 12) : Inport  Port=3
  ApGlobal In : Inport  Port=4
  RTOActive In : Inport  Port=5
  EngineKill In : Inport  Port=6
  AND : Logic  Inputs=3  IconShape=distinctive  AllPortsSameDT=off  OutDataTypeStr=boolean
  AND1 : Logic  IconShape=distinctive  AllPortsSameDT=off  OutDataTypeStr=boolean
  Compare To Constant : simulink/Logic and Bit Operations/Compare To Constant  relop=>=  const=10  OutDataTypeStr=boolean
  Compare To Constant1 : simulink/Logic and Bit Operations/Compare To Constant  relop=>=  const=11  OutDataTypeStr=boolean
  Compare To Constant2 : simulink/Logic and Bit Operations/Compare To Constant  relop===  const=11  OutDataTypeStr=boolean
  Compare To Constant3 : simulink/Logic and Bit Operations/Compare To Constant  relop=>=  const=RolloutElevTrigger  OutDataTypeStr=boolean
  Compare To Constant4 : simulink/Logic and Bit Operations/Compare To Constant  relop=>=  const=9  OutDataTypeStr=boolean
  Constant : Constant  Value=useFlareSlew
  Constant1 : Constant  Value=ThrottleMaxFlare
  Constant2 : Constant  Value=ThrottleMinRollout
  Constant3 : Constant  Value=ThrottleMinFlare
  Constant4 : Constant  Value=useElevatorKill
  Constant5 : Constant  Value=ThrottleRateRever
  Constant6 : Constant  Value=ThrottleRateRollout
  Constant7 : Constant  Value=ThrottleRateFlare
  Gain5 : Gain  Gain=-1
  Latch : Subsystem
  NOT1 : Logic  Operator=NOT  IconShape=distinctive  AllPortsSameDT=off  OutDataTypeStr=boolean
  OR : Logic  Operator=NOR  Inputs=3  IconShape=distinctive  AllPortsSameDT=off  OutDataTypeStr=boolean
  Rate Limiter : Subsystem
  Saturation Dynamic : simulink/Discontinuities/Saturation Dynamic  OutMin=[]  OutMax=[]  OutDataTypeStr=Inherit: Same as second input  OutDataType=fixdt(1, 16)  OutScaling=2^-10  DoSatur=off
  Switch{,1..5} (6 alike) : Switch  Criteria=u2 > Threshold
  Throttle Out : Outport
  wires:
  Constant2/1 -> Switch5/1, Switch/1
  Throttle In (0 - 100%)/1 -> Switch5/3, Switch3/3
  Switch5/1 -> Saturation Dynamic/2
  RTOActive In/1 -> OR/2
  ApGlobal In/1 -> NOT1/1
  OR/1 -> AND/3
  NOT1/1 -> OR/1
  Switch1/1 -> AND1/2
  Compare To Constant2/1 -> Switch1/3, AND1/1
  Switch4/1 -> Rate Limiter/1(up), Gain5/1  "OverridenTECSlewRate"
  AND/1 -> Switch3/2, Rate Limiter/4(Enable)  "flareSlewActive"
  Saturation Dynamic/1 -> Rate Limiter/2(u)
  Constant/1 -> AND/1
  Gain5/1 -> Rate Limiter/3(lo)
  Compare To Constant/1 -> AND/2
  AP Mode (0 - 12)/1 -> Compare To Constant/1, Compare To Constant4/1, Compare To Constant1/1, Compare To Constant2/1
  Switch3/1 -> Throttle Out/1
  Constant1/1 -> Saturation Dynamic/1
  Constant3/1 -> Switch/3
  Switch/1 -> Saturation Dynamic/3
  Piccolo Elevator In (deg.)/1 -> Compare To Constant3/1
  AND1/1 -> Switch5/2, Switch/2
  Constant4/1 -> Switch1/2
  Compare To Constant3/1 -> Switch1/1
  Rate Limiter/1(Y) -> Switch3/1
  Compare To Constant1/1 -> Switch4/2, Latch/1(D)
  Constant7/1 -> Switch2/3
  Constant6/1 -> Switch4/1
  Compare To Constant4/1 -> Latch/2(Enable/!Rst)
  Latch/1(Q_Latched) -> Switch2/2
  Constant5/1 -> Switch2/1
  Switch2/1 -> Switch4/3
  EngineKill In/1 -> OR/3

== system Lib_Piccolo/Throttle Control (Alt Mode)/LPF Energy Alpha ==
  Input : Inport
  Reset : Inport  Port=2
  Add1 : Sum  Commented=on  Inputs=++|
  Compare To Constant1 : simulink/Logic and Bit Operations/Compare To Constant  relop=>  const=0  OutDataTypeStr=uint8
  Compare To Constant2 : simulink/Logic and Bit Operations/Compare To Constant  Commented=on  relop=>  const=0  OutDataTypeStr=uint8
  Constant : Constant  Value=dt
  Constant1 : Constant  Value=EnergyBandwidth
  Constant11 : Constant  Commented=on  Value=EnergyBandwidth
  LPF Alpha Energy : MATLAB Function  TreatAsAtomicUnit=on
  Memory1 : Memory  InitialCondition=LPFenergyFFInit  InheritSampleTime=on  LinearizeAsDelay=on
  Switch1 : Switch  Commented=on  Criteria=u2 > Threshold
  Switch2 : Switch  Criteria=u2 > Threshold
  Unit Delay1 : UnitDelay  Commented=on  InitialCondition=LPFenergyFFInit  SampleTime=-1
  a1 : Gain  Commented=on  Gain=1-Fp_Energy2
  b0 : Gain  Commented=on  Gain=Fp_Energy2
  Output : Outport
  wires:
  Constant1/1 -> LPF Alpha Energy/4(bandwidth), Compare To Constant1/1
  Memory1/1 -> LPF Alpha Energy/1(xFiltOld)
  LPF Alpha Energy/1(xFilt) -> Switch2/1, Memory1/1
  Compare To Constant1/1 -> Switch2/2
  Input/1 -> Switch2/3, LPF Alpha Energy/3(xNew)
  Switch2/1 -> Output/1
  Constant/1 -> LPF Alpha Energy/2(dt)
  Unit Delay1/1 -> a1/1
  b0/1 -> Add1/2
  Compare To Constant2/1 -> Switch1/2
  a1/1 -> Add1/1
  Constant11/1 -> Compare To Constant2/1
  Add1/1 -> Switch1/1, Unit Delay1/1

== system Lib_Piccolo/Throttle Control (Alt Mode)/O//L Throttle Ramp ==
  Feedback Bus : Inport
  startFlag : Inport  Port=2
  Bus Selector : BusSelector  OutputSignals=Sim_VGround
  Constant : Constant  Value=0
  Constant4 : Constant  Value=ThrottleMax
  Constant5 : Constant  Value=SlowThrottleRate
  Constant6 : Constant  Value=FastThrottleRate
  Integrator1 : Integrator  ExternalReset=rising  InitialCondition=PrelaunchThrottle
  Switch : Switch  Criteria=u2 > Threshold
  Switch2 : Switch  Criteria=u2 > Threshold  Threshold=ThrottleSwitchSpeed
  Switch3 : Switch  Threshold=ThrottleMax
  Sim.LaunchThrottleCmd : Outport
  wires:
  Integrator1/1 -> Switch3/3, Switch3/2  "throttleIntegrator"
  Constant6/1 -> Switch2/1
  Switch3/1 -> Switch/1  "throttleSat"
  Constant4/1 -> Switch3/1
  Switch2/1 -> Integrator1/1
  Constant5/1 -> Switch2/3
  Bus Selector/1 -> Switch2/2  "<Sim_VGround>"
  Feedback Bus/1 -> Bus Selector/1
  startFlag/1 -> Integrator1/2, Switch/2  "throttleflag"
  Switch/1 -> Sim.LaunchThrottleCmd/1
  Constant/1 -> Switch/3

== system Lib_Piccolo/Throttle Control (Alt Mode)/Reset Conditions ==
  AP Mode : Inport
  Compare To Constant1 : simulink/Logic and Bit Operations/Compare To Constant  relop=<=  const=3.0  OutDataTypeStr=boolean
  NOT : Logic  Operator=NOT  IconShape=distinctive  AllPortsSameDT=off  OutDataTypeStr=boolean
  OR : Logic  Operator=OR  Inputs=3  IconShape=distinctive  AllPortsSameDT=off  OutDataTypeStr=boolean
  Reset : Outport
  wires:
  NOT/1 -> OR/1
  [Flag_TAS_Priority] -> OR/2
  Compare To Constant1/1 -> OR/3
  [ApGlobal] -> NOT/1
  OR/1 -> Reset/1
  AP Mode/1 -> Compare To Constant1/1

== system Lib_Piccolo/Throttle Control (Alt Mode)/Speed Flags ==
  Feedback Bus : Inport
  AND : Logic  IconShape=distinctive  AllPortsSameDT=off  OutDataTypeStr=boolean
  AND1 : Logic  IconShape=distinctive  AllPortsSameDT=off  OutDataTypeStr=boolean
  Bus Selector : BusSelector  OutputSignals=V_mps,apMode
  CAS2TAS : Subsystem
  CAS2TAS1 : Subsystem
  Compare To Constant : simulink/Logic and Bit Operations/Compare To Constant  relop=>=  const=4  OutDataTypeStr=boolean
  Constant : Constant  Value=IASmin
  Constant6 : Constant  Value=IASmax
  Less Than : RelationalOperator  Operator=<  OutDataTypeStr=boolean  RndMeth=Simplest
  Less Than1 : RelationalOperator  Operator=>  OutDataTypeStr=boolean  RndMeth=Simplest
  Flag_Underspeed : Outport
  Flag_Overspeed : Outport  Port=2
  wires:
  Bus Selector/2 -> Compare To Constant/1  "<apMode>"
  Bus Selector/1 -> Less Than1/1, Less Than/1  "<V_mps>"
  Less Than/1 -> AND/1
  CAS2TAS/1(TAS) -> Less Than/2
  Constant/1 -> CAS2TAS/2(CAS)
  Constant6/1 -> CAS2TAS1/2(CAS)
  CAS2TAS1/1(TAS) -> Less Than1/2
  Less Than1/1 -> AND1/2
  Feedback Bus/1 -> Bus Selector/1, CAS2TAS1/1(Feedback Bus), CAS2TAS/1(Feedback Bus)
  AND/1 -> Flag_Underspeed/1  "Flag_Underspeed"
  AND1/1 -> Flag_Overspeed/1  "Flag_Overspeed"
  Compare To Constant/1 -> AND1/1, AND/2

== system Lib_Piccolo/VRate Reference Selection/Alt Max Accel Rate Limit ==
  note: Y(k)
  note: U(k)
  up : Inport
  u : Inport  Port=2
  lo : Inport  Port=3
  Delay Input2 : UnitDelay  Description=Store in Global RAM  DisableCoverage=on  InitialCondition=RateLimitAltAccelInit  SampleTime=-1
  Difference Inputs1 : Sum  Description=Add in CPU  DisableCoverage=on  Inputs=+-  OutDataTypeStr=Inherit: Inherit via back propagation
  Difference Inputs2 : Sum  Description=Add in CPU  OutDataTypeStr=Inherit: Inherit via back propagation
  FixPt Data Type Duplicate : DataTypeDuplicate  DisableCoverage=on  NumInputPorts=7
  Saturation Dynamic2 : simulink/Discontinuities/Saturation Dynamic  OutMin=[]  OutMax=[]  OutDataTypeStr=Inherit: Same as second input  OutDataType=fixdt(1, 16)  OutScaling=2^-10  DoSatur=off
  delta fall limit : Product  DisableCoverage=on  Inputs=**  OutDataTypeStr=Inherit: Inherit via back propagation  SaturateOnIntegerOverflow=on
  delta rise limit : Product  DisableCoverage=on  Inputs=**  OutDataTypeStr=Inherit: Inherit via back propagation  SaturateOnIntegerOverflow=on
  sample time : SampleTimeMath  DisableCoverage=on  TsampMathOp=Ts Only  weightValue=1
  Y : Outport  InitialOutput=0
  wires:
  Difference Inputs2/1 -> Y/1, FixPt Data Type Duplicate/1, Delay Input2/1
  sample time/1 -> delta rise limit/2, delta fall limit/2
  Delay Input2/1 -> FixPt Data Type Duplicate/2, Difference Inputs1/2, Difference Inputs2/2  "Y(k-1)"
  up/1 -> delta rise limit/1
  u/1 -> sample time/1, FixPt Data Type Duplicate/5, Difference Inputs1/1
  Saturation Dynamic2/1 -> FixPt Data Type Duplicate/7, Difference Inputs2/1
  lo/1 -> delta fall limit/1
  delta rise limit/1 -> Saturation Dynamic2/1, FixPt Data Type Duplicate/6
  Difference Inputs1/1 -> Saturation Dynamic2/2, FixPt Data Type Duplicate/4  "( U(k) - Y(k-1) )"
  delta fall limit/1 -> Saturation Dynamic2/3, FixPt Data Type Duplicate/3
